simulink model "test_pgmanif"  (R2016b)
settings: Solver=FixedStepDiscrete  StartTime=0.0  StopTime=10.0  FixedStep=0.1  RelTol=1e-3
values from neighbouring files (symbols this model uses):
  A = eye(6)    [test_pgmanif_script.m]
  b = man_cart.id_element    [test_pgmanif_script.m]
  base = man_cyl.id_element    [test_pgmanif_script.m]
  base_s2r1 = man_sp.id_element    [test_pgmanif_script.m]
  covariance = eye(6)    [test_pgmanif_script.m]
  g = [1 0 0 1 0.707 0.707 0 0]'    [test_pgmanif_script.m]
  g_s2r1 = [1 0 0 1 0.707 0.707 0 0]'    [test_pgmanif_script.m]
  h = man_cyl.action(base, point, g)    [test_pgmanif_script.m]
  h_s2r1 = man_sp.action(base_s2r1, point_s2r1, g_s2r1)    [test_pgmanif_script.m]
  input = eye(6)    [test_pgmanif_script.m]
  input_s2r1 = eye(6)    [test_pgmanif_script.m]
  mu = man_cart.id_element    [test_pgmanif_script.m]
  point = man_cyl.exp(tangent, base)    [test_pgmanif_script.m]
  point_s2r1 = man_sp.exp(tangent_s2r1, base_s2r1)    [test_pgmanif_script.m]
  tangent = [0.1 0.1 0.1 0.1 0.1 0.1]'    [test_pgmanif_script.m]
  tangent_s2r1 = [0.1 0.1 0.1 0.1 0.1 0.1]'    [test_pgmanif_script.m]
undefined symbols (not defined in the file or in its folder): R1, R2, S2, SO2, SO3
libraries: pgmanif x14
settings Model: Creator=mueh_mm  LastModifiedBy=mueh_mm

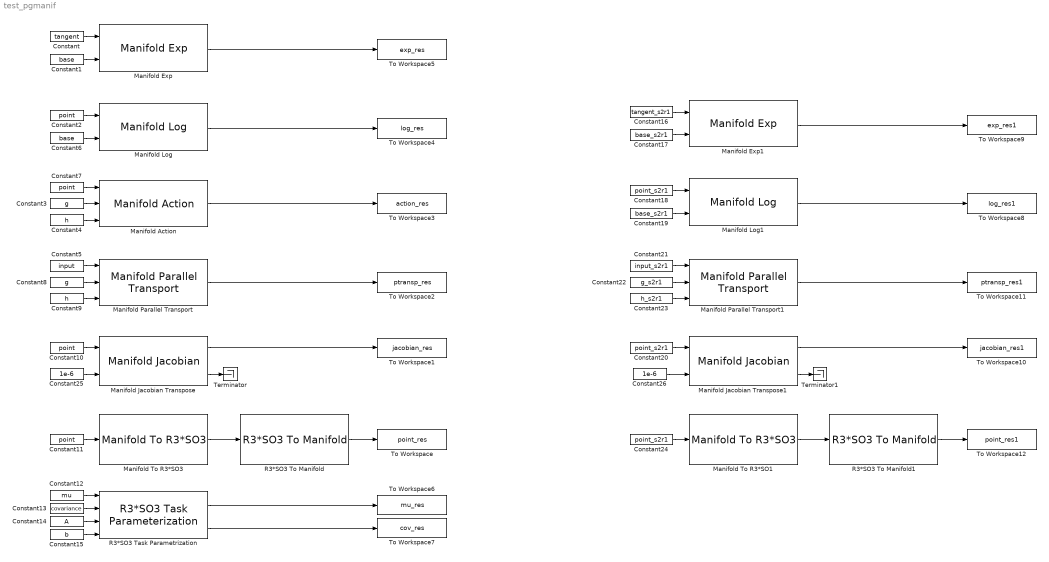
== system test_pgmanif ==
  Constant : Constant  Value=tangent
  Constant1 : Constant  Value=base
  Constant{2,7,10..11} (4 alike) : Constant  Value=point
  Constant12 : Constant  Value=mu
  Constant13 : Constant  Value=covariance
  Constant14 : Constant  Value=A
  Constant15 : Constant  Value=b
  Constant16 : Constant  Value=tangent_s2r1
  Constant17 : Constant  Value=base_s2r1
  Constant18 : Constant  Value=point_s2r1
  Constant19 : Constant  Value=base_s2r1
  Constant20 : Constant  Value=point_s2r1
  Constant21 : Constant  Value=input_s2r1
  Constant22 : Constant  Value=g_s2r1
  Constant23 : Constant  Value=h_s2r1
  Constant24 : Constant  Value=point_s2r1
  Constant25 : Constant  Value=1e-6
  Constant26 : Constant  Value=1e-6
  Constant3 : Constant  Value=g
  Constant4 : Constant  Value=h
  Constant5 : Constant  Value=input
  Constant6 : Constant  Value=base
  Constant8 : Constant  Value=g
  Constant9 : Constant  Value=h
  Manifold Action : pgmanif/Manifold Action  manifold_description_raw=SO2*R2*SO3  manifold_description=0  dim_manifold=0  dim_tangent=0
  Manifold Exp : pgmanif/Manifold Exp  manifold_description_raw=SO2*R2*SO3  manifold_description=0  dim_manifold=0  dim_tangent=0
  Manifold Exp1 : pgmanif/Manifold Exp  manifold_description_raw=S2*R1*SO3  manifold_description=0  dim_manifold=0  dim_tangent=0
  Manifold Jacobian Transpose : pgmanif/Manifold Jacobian  manifold_description_raw=SO2*R2*SO3  manifold_description=0  dim_manifold=0  dim_tangent=0  manifold_id=0
  Manifold Jacobian Transpose1 : pgmanif/Manifold Jacobian  manifold_description_raw=S2*R1*SO3  manifold_description=0  dim_manifold=0  dim_tangent=0  manifold_id=0
  Manifold Log : pgmanif/Manifold Log  manifold_description_raw=SO2*R2*SO3  manifold_description=0  dim_manifold=0  dim_tangent=0
  Manifold Log1 : pgmanif/Manifold Log  manifold_description_raw=S2*R1*SO3  manifold_description=0  dim_manifold=0  dim_tangent=0
  Manifold Parallel Transport : pgmanif/Manifold Parallel Transport  manifold_description_raw=SO2*R2*SO3  manifold_description=0  dim_manifold=0  dim_tangent=0
  Manifold Parallel Transport1 : pgmanif/Manifold Parallel Transport  manifold_description_raw=S2*R1*SO3  manifold_description=0  dim_manifold=0  dim_tangent=0
  Manifold To R3*SO1 : pgmanif/Manifold To R3*SO3  manifold_description_raw=S2*R1*SO3  manifold_description=0  dim_manifold=0  dim_tangent=0
  Manifold To R3*SO3 : pgmanif/Manifold To R3*SO3  manifold_description_raw=SO2*R2*SO3  manifold_description=0  dim_manifold=0  dim_tangent=0
  R3*SO3 Task Parametrization : pgmanif/R3*SO3 Task Parameterization  dim_tangent=0  dim_manifold=0
  R3*SO3 To Manifold : pgmanif/R3*SO3 To Manifold  manifold_description_raw=SO2*R2*SO3  manifold_description=0  dim_manifold=0  dim_tangent=0
  R3*SO3 To Manifold1 : pgmanif/R3*SO3 To Manifold  manifold_description_raw=S2*R1*SO3  manifold_description=0  dim_manifold=0  dim_tangent=0
  Terminator : Terminator
  Terminator1 : Terminator
  To Workspace : ToWorkspace  VariableName=point_res  SaveFormat=Timeseries  SampleTime=-1
  To Workspace1 : ToWorkspace  VariableName=jacobian_res  SaveFormat=Timeseries  SampleTime=-1
  To Workspace10 : ToWorkspace  VariableName=jacobian_res1  SaveFormat=Timeseries  SampleTime=-1
  To Workspace11 : ToWorkspace  VariableName=ptransp_res1  SaveFormat=Timeseries  SampleTime=-1
  To Workspace12 : ToWorkspace  VariableName=point_res1  SaveFormat=Timeseries  SampleTime=-1
  To Workspace2 : ToWorkspace  VariableName=ptransp_res  SaveFormat=Timeseries  SampleTime=-1
  To Workspace3 : ToWorkspace  VariableName=action_res  SaveFormat=Timeseries  SampleTime=-1
  To Workspace4 : ToWorkspace  VariableName=log_res  SaveFormat=Timeseries  SampleTime=-1
  To Workspace5 : ToWorkspace  VariableName=exp_res  SaveFormat=Timeseries  SampleTime=-1
  To Workspace6 : ToWorkspace  VariableName=mu_res  SaveFormat=Timeseries  SampleTime=-1
  To Workspace7 : ToWorkspace  VariableName=cov_res  SaveFormat=Timeseries  SampleTime=-1
  To Workspace8 : ToWorkspace  VariableName=log_res1  SaveFormat=Timeseries  SampleTime=-1
  To Workspace9 : ToWorkspace  VariableName=exp_res1  SaveFormat=Timeseries  SampleTime=-1
  wires:
  Constant/1 -> Manifold Exp/1
  Constant1/1 -> Manifold Exp/2
  Constant6/1 -> Manifold Log/2
  Constant2/1 -> Manifold Log/1
  Constant7/1 -> Manifold Action/1
  Constant3/1 -> Manifold Action/2
  Constant4/1 -> Manifold Action/3
  Constant5/1 -> Manifold Parallel Transport/1
  Constant8/1 -> Manifold Parallel Transport/2
  Constant9/1 -> Manifold Parallel Transport/3
  Constant10/1 -> Manifold Jacobian Transpose/1
  Constant11/1 -> Manifold To R3*SO3/1
  Manifold To R3*SO3/1 -> R3*SO3 To Manifold/1
  Constant12/1 -> R3*SO3 Task Parametrization/1
  Constant14/1 -> R3*SO3 Task Parametrization/3
  Constant15/1 -> R3*SO3 Task Parametrization/4
  Constant13/1 -> R3*SO3 Task Parametrization/2
  R3*SO3 To Manifold/1 -> To Workspace/1
  Manifold Jacobian Transpose/1 -> To Workspace1/1
  Manifold Parallel Transport/1 -> To Workspace2/1
  Manifold Action/1 -> To Workspace3/1
  Manifold Log/1 -> To Workspace4/1
  Manifold Exp/1 -> To Workspace5/1
  R3*SO3 Task Parametrization/1 -> To Workspace6/1
  R3*SO3 Task Parametrization/2 -> To Workspace7/1
  Constant16/1 -> Manifold Exp1/1
  Constant17/1 -> Manifold Exp1/2
  Constant19/1 -> Manifold Log1/2
  Constant18/1 -> Manifold Log1/1
  Manifold Log1/1 -> To Workspace8/1
  Manifold Exp1/1 -> To Workspace9/1
  Constant21/1 -> Manifold Parallel Transport1/1
  Constant22/1 -> Manifold Parallel Transport1/2
  Constant23/1 -> Manifold Parallel Transport1/3
  Constant20/1 -> Manifold Jacobian Transpose1/1
  Manifold Jacobian Transpose1/1 -> To Workspace10/1
  Manifold Parallel Transport1/1 -> To Workspace11/1
  Constant24/1 -> Manifold To R3*SO1/1
  Manifold To R3*SO1/1 -> R3*SO3 To Manifold1/1
  R3*SO3 To Manifold1/1 -> To Workspace12/1
  Constant25/1 -> Manifold Jacobian Transpose/2
  Manifold Jacobian Transpose/2 -> Terminator/1
  Constant26/1 -> Manifold Jacobian Transpose1/2
  Manifold Jacobian Transpose1/2 -> Terminator1/1
